simulink model "Model"  (R2021a)
settings: Solver=VariableStepAuto  StartTime=0.0  StopTime=8  RelTol=1e-3  AbsTol=1e-3
settings Model: Creator=Basa Sidvik  LastModifiedBy=Basa Sidvik
settings SolverCC: AutoScaleAbsTol=off  AlgebraicLoopSolver=TrustRegion
settings DebuggingCC: SymbolicDimsDataTypeCodeGenerationDiagnostic=none  SFMachineParentedDataDiag=warning
settings SFSimCC: CustomCodeUndefinedFunction=UseInterfaceOnly
settings SimscapeCC: SimscapeLogType=all  SimscapeLogSimulationStatistics=on  SimscapeLogDataHistory=10000

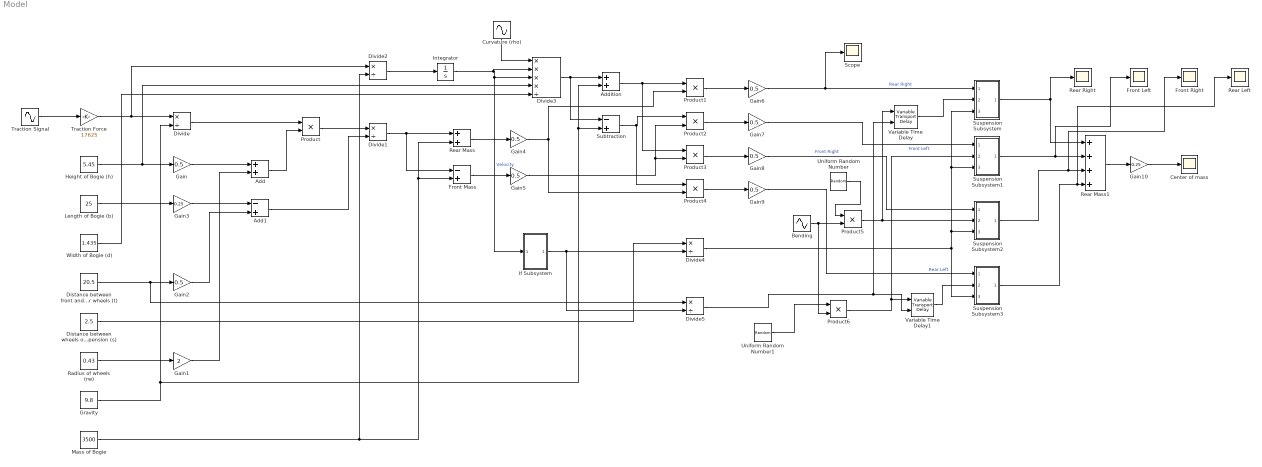
== system Model ==
  Add : Sum
  Add1 : Sum  Inputs=-+
  Addition : Sum
  Bending : Sin  Amplitude=0.004  SampleTime=0
  Center of mass : Scope
  Curvature (rho) : Sin  Amplitude=0.0004  SampleTime=0
  Distance between front and rear wheels (t) : Constant  Value=20.5
  Distance between wheels of same suspension (s) : Constant  Value=2.5
  Divide{,1..2,4..5} (5 alike) : Product  Inputs=*/
  Divide3 : Product  Inputs=****/
  Front Left : Scope
  Front Mass : Sum  Inputs=-+
  Front Right : Scope
  Gain{,2,4..9} (8 alike) : Gain  Gain=0.5
  Gain1 : Gain  Gain=2
  Gain10 : Gain  Gain=0.25
  Gain3 : Gain  Gain=0.25
  Gravity : Constant  Value=9.8
  Height of Bogie (h) : Constant  Value=5.45
  If Subsystem : Subsystem
  Integrator : Integrator
  Length of Bogie (b) : Constant  Value=25
  Mass of Bogie : Constant  Value=3500
  Product{,1..6} (7 alike) : Product
  Radius of wheels (rw) : Constant  Value=0.43
  Rear Left : Scope
  Rear Mass : Sum
  Rear Mass1 : Sum  Inputs=++++
  Rear Right : Scope
  Scope : Scope
  Subtraction : Sum  Inputs=-+
  Suspension Subsystem : Subsystem
  Suspension Subsystem1 : Subsystem
  Suspension Subsystem2 : Subsystem
  Suspension Subsystem3 : Subsystem
  Traction Force : Gain  Gain=17625
  Traction Signal : Sin  Frequency=0.01  SampleTime=0
  Uniform Random Number : UniformRandomNumber  Minimum=-0.001  Maximum=0.001  SampleTime=0.1
  Uniform Random Number1 : UniformRandomNumber  Minimum=-0.001  Maximum=0.001  SampleTime=0.001
  Variable Time Delay : VariableTransportDelay  MaximumDelay=1000000
  Variable Time Delay1 : VariableTransportDelay  MaximumDelay=1000000
  Width of Bogie (d) : Constant  Value=1.435
  wires:
  Traction Signal/1 -> Traction Force/1
  Traction Force/1 -> Divide2/1, Divide/1
  Height of Bogie (h)/1 -> Divide3/4, Gain/1
  Radius of wheels (rw)/1 -> Gain1/1
  Gain/1 -> Add/1
  Gain1/1 -> Add/2
  Divide/1 -> Product/1
  Add/1 -> Product/2
  Distance between front and rear wheels (t)/1 -> Divide5/1, Gain2/1
  Length of Bogie (b)/1 -> Gain3/1
  Gain3/1 -> Add1/1
  Gain2/1 -> Add1/2
  Product/1 -> Divide1/1
  Add1/1 -> Divide1/2
  Divide1/1 -> Front Mass/1, Rear Mass/1
  Mass of Bogie/1 -> Divide2/2, Front Mass/2, Rear Mass/2
  Rear Mass/1 -> Gain4/1
  Front Mass/1 -> Gain5/1
  Divide2/1 -> Integrator/1
  Integrator/1 -> Divide3/2, If Subsystem/1(In1), Divide3/3  "Velocity"
  Curvature (rho)/1 -> Divide3/1
  Width of Bogie (d)/1 -> Divide3/5
  Divide3/1 -> Subtraction/1, Addition/1
  Gravity/1 -> Subtraction/2, Addition/2, Divide/2
  Addition/1 -> Product3/1, Product1/1
  Product1/1 -> Gain6/1
  Gain4/1 -> Product4/2, Product1/2
  Product2/1 -> Gain7/1
  Product3/1 -> Gain8/1
  Product4/1 -> Gain9/1
  Gain5/1 -> Product3/2, Product2/2
  Subtraction/1 -> Product4/1, Product2/1
  Gain6/1 -> Scope/1, Suspension Subsystem/1(In1)  "Rear Right"
  Gain7/1 -> Suspension Subsystem1/1(In1)  "Front Left"
  Gain8/1 -> Suspension Subsystem2/1(In1)  "Front Right"
  Gain9/1 -> Suspension Subsystem3/1(In1)  "Rear Left"
  Variable Time Delay/1 -> Suspension Subsystem/2(In2)
  Suspension Subsystem/1(Out1) -> Rear Mass1/1, Rear Right/1
  Distance between wheels of same suspension (s)/1 -> Divide4/1
  Divide4/1 -> Suspension Subsystem3/3(In3), Suspension Subsystem2/3(In3), Suspension Subsystem1/3(In3), Suspension Subsystem/3(In3)
  Product5/1 -> Suspension Subsystem2/2(In2), Variable Time Delay/1
  Product6/1 -> Suspension Subsystem1/2(In2), Variable Time Delay1/1
  Variable Time Delay1/1 -> Suspension Subsystem3/2(In2)
  Divide5/1 -> Variable Time Delay1/2, Variable Time Delay/2
  Suspension Subsystem1/1(Out1) -> Front Left/1, Rear Mass1/2
  Suspension Subsystem2/1(Out1) -> Front Right/1, Rear Mass1/3
  Suspension Subsystem3/1(Out1) -> Rear Left/1, Rear Mass1/4
  Rear Mass1/1 -> Gain10/1
  Gain10/1 -> Center of mass/1
  Bending/1 -> Product6/2, Product5/2
  Uniform Random Number/1 -> Product5/1
  Uniform Random Number1/1 -> Product6/1
  If Subsystem/1(Out1) -> Divide5/2, Divide4/2

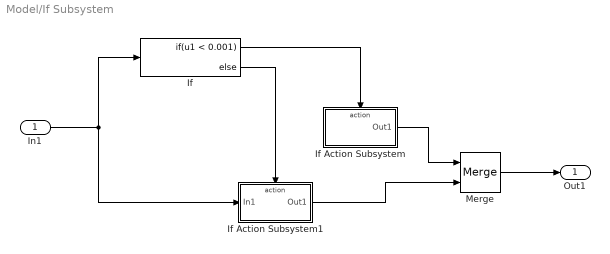
== system Model/If Subsystem ==
  In1 : Inport
  If : If  IfExpression=u1 < 0.001
  If Action Subsystem : Subsystem  TreatAsAtomicUnit=on
  If Action Subsystem1 : Subsystem  TreatAsAtomicUnit=on
  Merge : Merge
  Out1 : Outport
  wires:
  In1/1 -> If Action Subsystem1/1(In1), If/1
  If/2 -> If Action Subsystem1/Action
  If Action Subsystem1/1(Out1) -> Merge/2
  Merge/1 -> Out1/1
  If Action Subsystem/1(Out1) -> Merge/1
  If/1 -> If Action Subsystem/Action

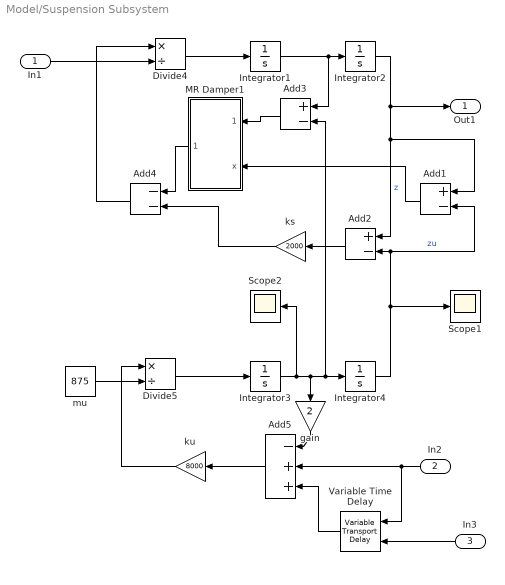
== system Model/Suspension Subsystem ==
  In1 : Inport
  In2 : Inport  Port=2
  In3 : Inport  Port=3
  Add1 : Sum  Inputs=+-
  Add2 : Sum  Inputs=+-
  Add3 : Sum  Inputs=+-
  Add4 : Sum  Inputs=--
  Add5 : Sum  Inputs=-++
  Divide4 : Product  Inputs=*/
  Divide5 : Product  Inputs=*/
  Integrator{1..4} (4 alike) : Integrator
  MR Damper1 : Subsystem
  Scope1 : Scope
  Scope2 : Scope
  Variable Time Delay : VariableTransportDelay  MaximumDelay=1e6
  gain : Gain  Gain=2
  ks : Gain  Gain=2000
  ku : Gain  Gain=8000
  mu : Constant  Value=875
  Out1 : Outport
  wires:
  Integrator4/1 -> Add1/2, Add2/2, Scope1/1  "zu"
  Integrator2/1 -> Out1/1, Add2/1, Add1/1  "z"
  Integrator1/1 -> Add3/1, Integrator2/1
  Integrator3/1 -> Scope2/1, gain/1, Add3/2, Integrator4/1
  Divide4/1 -> Integrator1/1
  In2/1 -> Variable Time Delay/1, Add5/2
  ku/1 -> Divide5/1
  Add2/1 -> ks/1
  Divide5/1 -> Integrator3/1
  mu/1 -> Divide5/2
  Add5/1 -> ku/1
  Add3/1 -> MR Damper1/1(xdot)
  Add4/1 -> Divide4/1
  MR Damper1/1(Force) -> Add4/1
  In1/1 -> Divide4/2
  Variable Time Delay/1 -> Add5/3
  ks/1 -> Add4/2
  In3/1 -> Variable Time Delay/2
  Add1/1 -> MR Damper1/2(x)
  gain/1 -> Add5/1

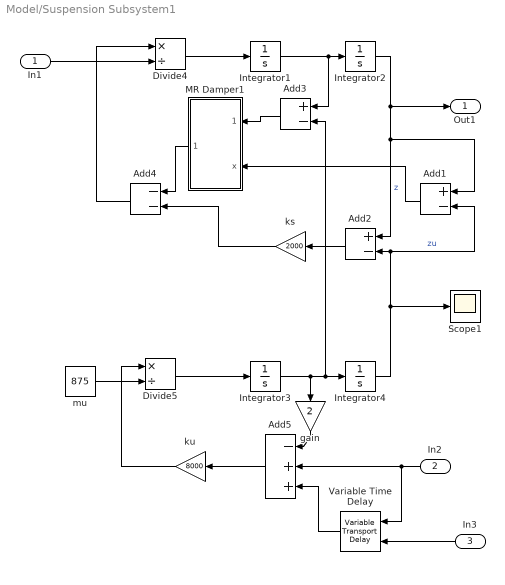
== system Model/Suspension Subsystem1 ==
  In1 : Inport
  In2 : Inport  Port=2
  In3 : Inport  Port=3
  Add1 : Sum  Inputs=+-
  Add2 : Sum  Inputs=+-
  Add3 : Sum  Inputs=+-
  Add4 : Sum  Inputs=--
  Add5 : Sum  Inputs=-++
  Divide4 : Product  Inputs=*/
  Divide5 : Product  Inputs=*/
  Integrator{1..4} (4 alike) : Integrator
  MR Damper1 : Subsystem
  Scope1 : Scope
  Variable Time Delay : VariableTransportDelay  MaximumDelay=1e6
  gain : Gain  Gain=2
  ks : Gain  Gain=2000
  ku : Gain  Gain=8000
  mu : Constant  Value=875
  Out1 : Outport
  wires:
  Integrator4/1 -> Add1/2, Add2/2, Scope1/1  "zu"
  Integrator2/1 -> Out1/1, Add2/1, Add1/1  "z"
  Integrator1/1 -> Add3/1, Integrator2/1
  Integrator3/1 -> gain/1, Add3/2, Integrator4/1
  Divide4/1 -> Integrator1/1
  In2/1 -> Variable Time Delay/1, Add5/2
  ku/1 -> Divide5/1
  Add2/1 -> ks/1
  Divide5/1 -> Integrator3/1
  mu/1 -> Divide5/2
  Add5/1 -> ku/1
  Add3/1 -> MR Damper1/1(xdot)
  Add4/1 -> Divide4/1
  MR Damper1/1(Force) -> Add4/1
  In1/1 -> Divide4/2
  Variable Time Delay/1 -> Add5/3
  ks/1 -> Add4/2
  In3/1 -> Variable Time Delay/2
  Add1/1 -> MR Damper1/2(x)
  gain/1 -> Add5/1

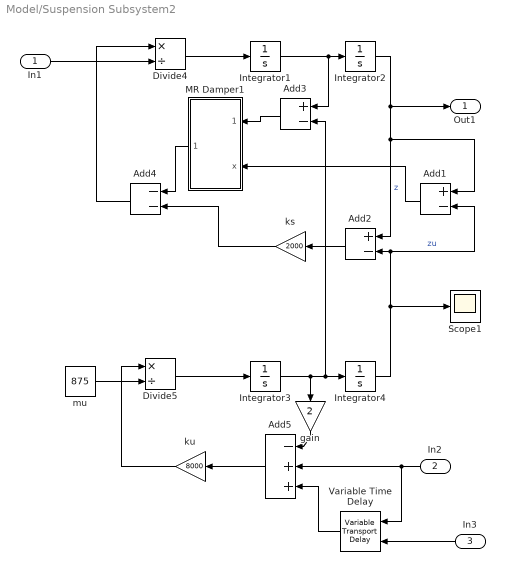
== system Model/Suspension Subsystem2 ==
  In1 : Inport
  In2 : Inport  Port=2
  In3 : Inport  Port=3
  Add1 : Sum  Inputs=+-
  Add2 : Sum  Inputs=+-
  Add3 : Sum  Inputs=+-
  Add4 : Sum  Inputs=--
  Add5 : Sum  Inputs=-++
  Divide4 : Product  Inputs=*/
  Divide5 : Product  Inputs=*/
  Integrator{1..4} (4 alike) : Integrator
  MR Damper1 : Subsystem
  Scope1 : Scope
  Variable Time Delay : VariableTransportDelay  MaximumDelay=1e6
  gain : Gain  Gain=2
  ks : Gain  Gain=2000
  ku : Gain  Gain=8000
  mu : Constant  Value=875
  Out1 : Outport
  wires:
  Integrator4/1 -> Add1/2, Add2/2, Scope1/1  "zu"
  Integrator2/1 -> Out1/1, Add2/1, Add1/1  "z"
  Integrator1/1 -> Add3/1, Integrator2/1
  Integrator3/1 -> gain/1, Add3/2, Integrator4/1
  Divide4/1 -> Integrator1/1
  In2/1 -> Variable Time Delay/1, Add5/2
  ku/1 -> Divide5/1
  Add2/1 -> ks/1
  Divide5/1 -> Integrator3/1
  mu/1 -> Divide5/2
  Add5/1 -> ku/1
  Add3/1 -> MR Damper1/1(xdot)
  Add4/1 -> Divide4/1
  MR Damper1/1(Force) -> Add4/1
  In1/1 -> Divide4/2
  Variable Time Delay/1 -> Add5/3
  ks/1 -> Add4/2
  In3/1 -> Variable Time Delay/2
  Add1/1 -> MR Damper1/2(x)
  gain/1 -> Add5/1

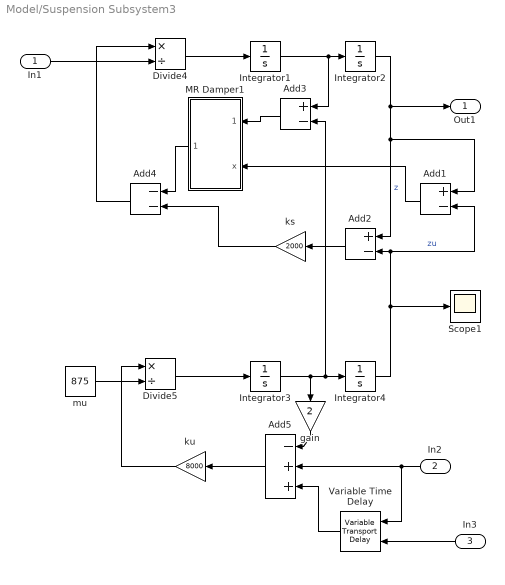
== system Model/Suspension Subsystem3 ==
  In1 : Inport
  In2 : Inport  Port=2
  In3 : Inport  Port=3
  Add1 : Sum  Inputs=+-
  Add2 : Sum  Inputs=+-
  Add3 : Sum  Inputs=+-
  Add4 : Sum  Inputs=--
  Add5 : Sum  Inputs=-++
  Divide4 : Product  Inputs=*/
  Divide5 : Product  Inputs=*/
  Integrator{1..4} (4 alike) : Integrator
  MR Damper1 : Subsystem
  Scope1 : Scope
  Variable Time Delay : VariableTransportDelay  MaximumDelay=1e6
  gain : Gain  Gain=2
  ks : Gain  Gain=2000
  ku : Gain  Gain=8000
  mu : Constant  Value=875
  Out1 : Outport
  wires:
  Integrator4/1 -> Add1/2, Add2/2, Scope1/1  "zu"
  Integrator2/1 -> Out1/1, Add2/1, Add1/1  "z"
  Integrator1/1 -> Add3/1, Integrator2/1
  Integrator3/1 -> gain/1, Add3/2, Integrator4/1
  Divide4/1 -> Integrator1/1
  In2/1 -> Variable Time Delay/1, Add5/2
  ku/1 -> Divide5/1
  Add2/1 -> ks/1
  Divide5/1 -> Integrator3/1
  mu/1 -> Divide5/2
  Add5/1 -> ku/1
  Add3/1 -> MR Damper1/1(xdot)
  Add4/1 -> Divide4/1
  MR Damper1/1(Force) -> Add4/1
  In1/1 -> Divide4/2
  Variable Time Delay/1 -> Add5/3
  ks/1 -> Add4/2
  In3/1 -> Variable Time Delay/2
  Add1/1 -> MR Damper1/2(x)
  gain/1 -> Add5/1

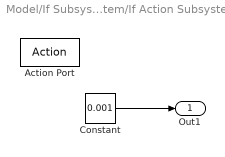
== system Model/If Subsystem/If Action Subsystem ==
  Action Port : ActionPort  ActionPortLabel=if(u1 < 0.001)
  Constant : Constant  Value=0.001
  Out1 : Outport
  wires:
  Constant/1 -> Out1/1

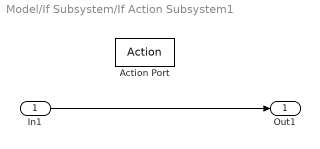
== system Model/If Subsystem/If Action Subsystem1 ==
  In1 : Inport
  Action Port : ActionPort  ActionPortLabel=else
  Out1 : Outport
  wires:
  In1/1 -> Out1/1

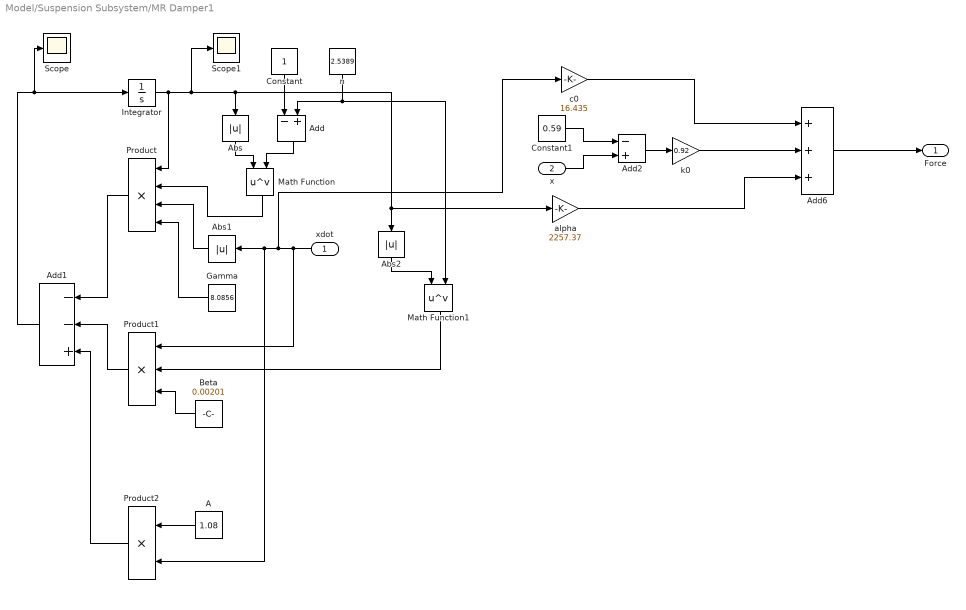
== system Model/Suspension Subsystem/MR Damper1 ==
  xdot : Inport
  x : Inport  Port=2
  A : Constant  Value=1.08
  Abs : Abs
  Abs1 : Abs
  Abs2 : Abs
  Add : Sum  Inputs=-+
  Add1 : Sum  Inputs=--+  OutMin=[-1000000]  OutMax=[1000000]
  Add2 : Sum  Inputs=-+
  Add6 : Sum  Inputs=+++
  Beta : Constant  Value=0.00201
  Constant : Constant
  Constant1 : Constant  Value=0.59
  Gamma : Constant  Value=8.0856
  Integrator : Integrator  LimitOutput=on  AbsoluteTolerance=1e6
  Math Function : Math  Operator=pow  OutputSignalType=real  SaturateOnIntegerOverflow=on
  Math Function1 : Math  Operator=pow  OutputSignalType=real  SaturateOnIntegerOverflow=on
  Product : Product  Inputs=4
  Product1 : Product  Inputs=3
  Product2 : Product
  Scope : Scope
  Scope1 : Scope
  alpha : Gain  Gain=2257.37
  c0 : Gain  Gain=16.435
  k0 : Gain  Gain=0.92
  n : Constant  Value=2.5389
  Force : Outport
  wires:
  Integrator/1 -> Scope1/1, Abs2/1, alpha/1, Abs/1, Product/1
  k0/1 -> Add6/2
  alpha/1 -> Add6/3
  Add/1 -> Math Function/2
  Gamma/1 -> Product/4
  Constant/1 -> Add/1
  xdot/1 -> c0/1, Abs1/1, Product2/2, Product1/1
  Math Function/1 -> Product/2
  A/1 -> Product2/1
  Add1/1 -> Scope/1, Integrator/1
  Beta/1 -> Product1/3
  Abs1/1 -> Product/3
  n/1 -> Math Function1/2, Add/2
  Abs/1 -> Math Function/1
  Abs2/1 -> Math Function1/1
  Product1/1 -> Add1/2
  Add6/1 -> Force/1
  Product2/1 -> Add1/3
  c0/1 -> Add6/1
  Product/1 -> Add1/1
  Math Function1/1 -> Product1/2
  x/1 -> Add2/2
  Constant1/1 -> Add2/1
  Add2/1 -> k0/1

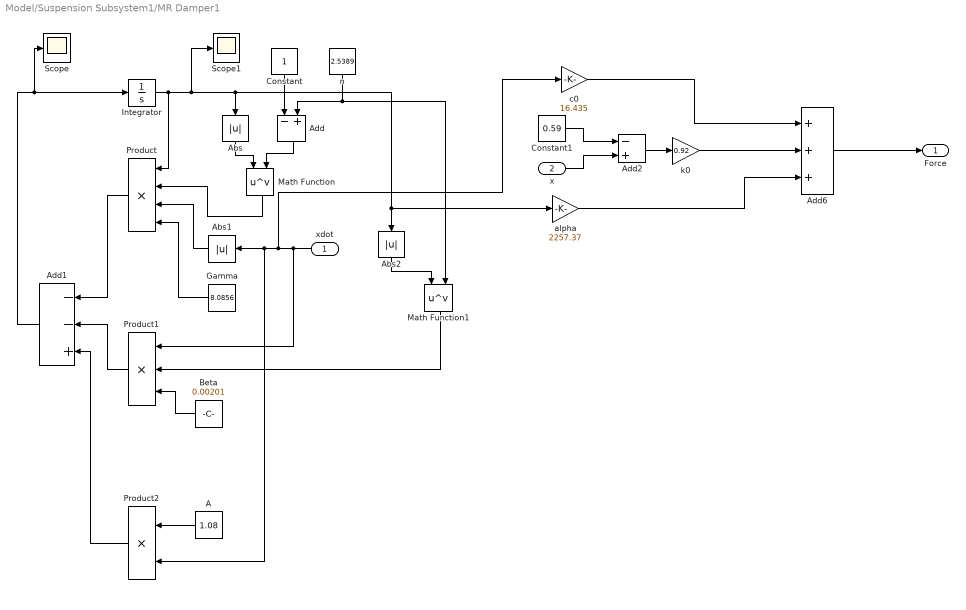
== system Model/Suspension Subsystem1/MR Damper1 ==
  xdot : Inport
  x : Inport  Port=2
  A : Constant  Value=1.08
  Abs : Abs
  Abs1 : Abs
  Abs2 : Abs
  Add : Sum  Inputs=-+
  Add1 : Sum  Inputs=--+  OutMin=[-1000000]  OutMax=[1000000]
  Add2 : Sum  Inputs=-+
  Add6 : Sum  Inputs=+++
  Beta : Constant  Value=0.00201
  Constant : Constant
  Constant1 : Constant  Value=0.59
  Gamma : Constant  Value=8.0856
  Integrator : Integrator  LimitOutput=on  AbsoluteTolerance=1e6
  Math Function : Math  Operator=pow  OutputSignalType=real  SaturateOnIntegerOverflow=on
  Math Function1 : Math  Operator=pow  OutputSignalType=real  SaturateOnIntegerOverflow=on
  Product : Product  Inputs=4
  Product1 : Product  Inputs=3
  Product2 : Product
  Scope : Scope
  Scope1 : Scope
  alpha : Gain  Gain=2257.37
  c0 : Gain  Gain=16.435
  k0 : Gain  Gain=0.92
  n : Constant  Value=2.5389
  Force : Outport
  wires:
  Integrator/1 -> Scope1/1, Abs2/1, alpha/1, Abs/1, Product/1
  k0/1 -> Add6/2
  alpha/1 -> Add6/3
  Add/1 -> Math Function/2
  Gamma/1 -> Product/4
  Constant/1 -> Add/1
  xdot/1 -> c0/1, Abs1/1, Product2/2, Product1/1
  Math Function/1 -> Product/2
  A/1 -> Product2/1
  Add1/1 -> Scope/1, Integrator/1
  Beta/1 -> Product1/3
  Abs1/1 -> Product/3
  n/1 -> Math Function1/2, Add/2
  Abs/1 -> Math Function/1
  Abs2/1 -> Math Function1/1
  Product1/1 -> Add1/2
  Add6/1 -> Force/1
  Product2/1 -> Add1/3
  c0/1 -> Add6/1
  Product/1 -> Add1/1
  Math Function1/1 -> Product1/2
  x/1 -> Add2/2
  Constant1/1 -> Add2/1
  Add2/1 -> k0/1

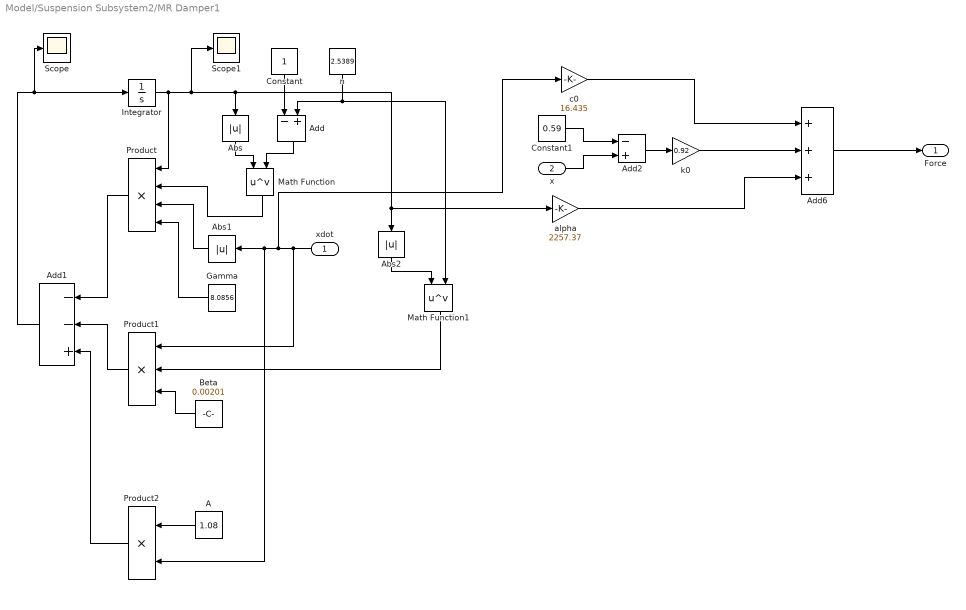
== system Model/Suspension Subsystem2/MR Damper1 ==
  xdot : Inport
  x : Inport  Port=2
  A : Constant  Value=1.08
  Abs : Abs
  Abs1 : Abs
  Abs2 : Abs
  Add : Sum  Inputs=-+
  Add1 : Sum  Inputs=--+  OutMin=[-1000000]  OutMax=[1000000]
  Add2 : Sum  Inputs=-+
  Add6 : Sum  Inputs=+++
  Beta : Constant  Value=0.00201
  Constant : Constant
  Constant1 : Constant  Value=0.59
  Gamma : Constant  Value=8.0856
  Integrator : Integrator  LimitOutput=on  AbsoluteTolerance=1e6
  Math Function : Math  Operator=pow  OutputSignalType=real  SaturateOnIntegerOverflow=on
  Math Function1 : Math  Operator=pow  OutputSignalType=real  SaturateOnIntegerOverflow=on
  Product : Product  Inputs=4
  Product1 : Product  Inputs=3
  Product2 : Product
  Scope : Scope
  Scope1 : Scope
  alpha : Gain  Gain=2257.37
  c0 : Gain  Gain=16.435
  k0 : Gain  Gain=0.92
  n : Constant  Value=2.5389
  Force : Outport
  wires:
  Integrator/1 -> Scope1/1, Abs2/1, alpha/1, Abs/1, Product/1
  k0/1 -> Add6/2
  alpha/1 -> Add6/3
  Add/1 -> Math Function/2
  Gamma/1 -> Product/4
  Constant/1 -> Add/1
  xdot/1 -> c0/1, Abs1/1, Product2/2, Product1/1
  Math Function/1 -> Product/2
  A/1 -> Product2/1
  Add1/1 -> Scope/1, Integrator/1
  Beta/1 -> Product1/3
  Abs1/1 -> Product/3
  n/1 -> Math Function1/2, Add/2
  Abs/1 -> Math Function/1
  Abs2/1 -> Math Function1/1
  Product1/1 -> Add1/2
  Add6/1 -> Force/1
  Product2/1 -> Add1/3
  c0/1 -> Add6/1
  Product/1 -> Add1/1
  Math Function1/1 -> Product1/2
  x/1 -> Add2/2
  Constant1/1 -> Add2/1
  Add2/1 -> k0/1

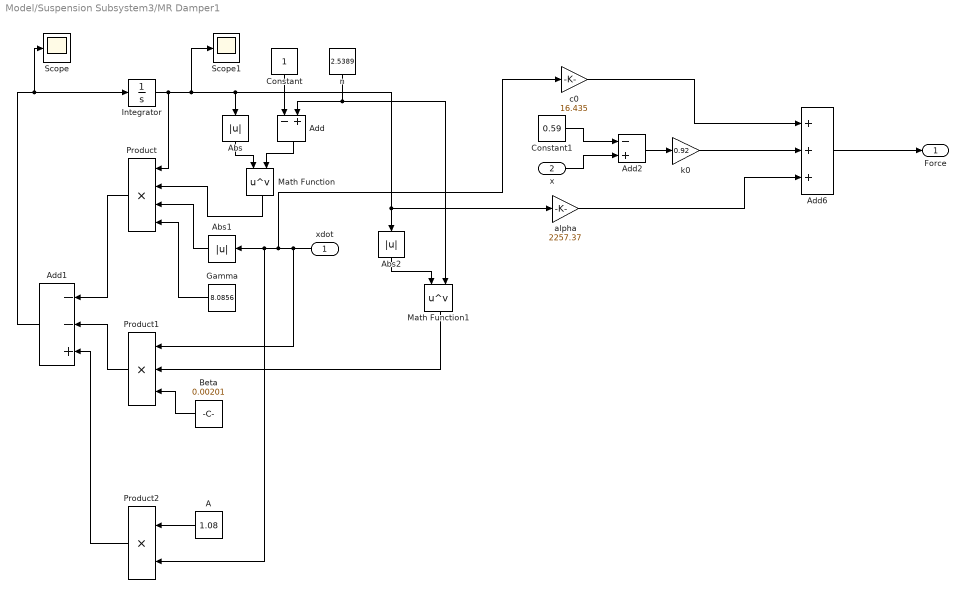
== system Model/Suspension Subsystem3/MR Damper1 ==
  xdot : Inport
  x : Inport  Port=2
  A : Constant  Value=1.08
  Abs : Abs
  Abs1 : Abs
  Abs2 : Abs
  Add : Sum  Inputs=-+
  Add1 : Sum  Inputs=--+  OutMin=[-1000000]  OutMax=[1000000]
  Add2 : Sum  Inputs=-+
  Add6 : Sum  Inputs=+++
  Beta : Constant  Value=0.00201
  Constant : Constant
  Constant1 : Constant  Value=0.59
  Gamma : Constant  Value=8.0856
  Integrator : Integrator  LimitOutput=on  AbsoluteTolerance=1e6
  Math Function : Math  Operator=pow  OutputSignalType=real  SaturateOnIntegerOverflow=on
  Math Function1 : Math  Operator=pow  OutputSignalType=real  SaturateOnIntegerOverflow=on
  Product : Product  Inputs=4
  Product1 : Product  Inputs=3
  Product2 : Product
  Scope : Scope
  Scope1 : Scope
  alpha : Gain  Gain=2257.37
  c0 : Gain  Gain=16.435
  k0 : Gain  Gain=0.92
  n : Constant  Value=2.5389
  Force : Outport
  wires:
  Integrator/1 -> Scope1/1, Abs2/1, alpha/1, Abs/1, Product/1
  k0/1 -> Add6/2
  alpha/1 -> Add6/3
  Add/1 -> Math Function/2
  Gamma/1 -> Product/4
  Constant/1 -> Add/1
  xdot/1 -> c0/1, Abs1/1, Product2/2, Product1/1
  Math Function/1 -> Product/2
  A/1 -> Product2/1
  Add1/1 -> Scope/1, Integrator/1
  Beta/1 -> Product1/3
  Abs1/1 -> Product/3
  n/1 -> Math Function1/2, Add/2
  Abs/1 -> Math Function/1
  Abs2/1 -> Math Function1/1
  Product1/1 -> Add1/2
  Add6/1 -> Force/1
  Product2/1 -> Add1/3
  c0/1 -> Add6/1
  Product/1 -> Add1/1
  Math Function1/1 -> Product1/2
  x/1 -> Add2/2
  Constant1/1 -> Add2/1
  Add2/1 -> k0/1
